simulink model "task5_simulink"  (R2026a)
settings: Solver=VariableStepAuto  StopTime=2
values from neighbouring files (symbols this model uses):
  k = transition_idx(j)    [task4.m]    (also in task5.m = k_values(i); task5_original.m = k_values(i))
  K = place(A, B, desired_poles)    [task3.m]    (also in task4.m; task5.m; task5_original.m)
  x0 = initial_conditions(i,:)'    [task4.m]    (also in task5.m = [0; task5_original.m = [0)
settings Model: Creator=DELL  LastModifiedBy=DELL

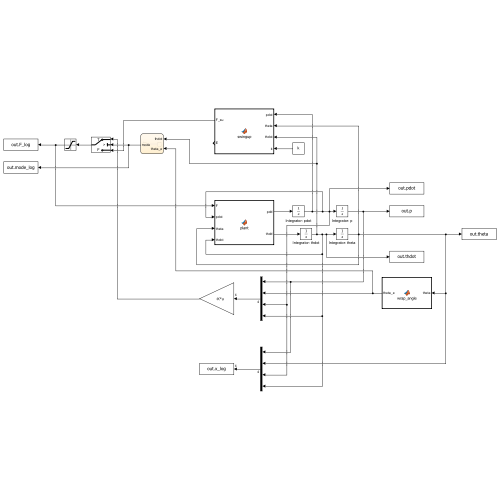
[thumbnail: Simulink's stored preview of the top-level diagram]
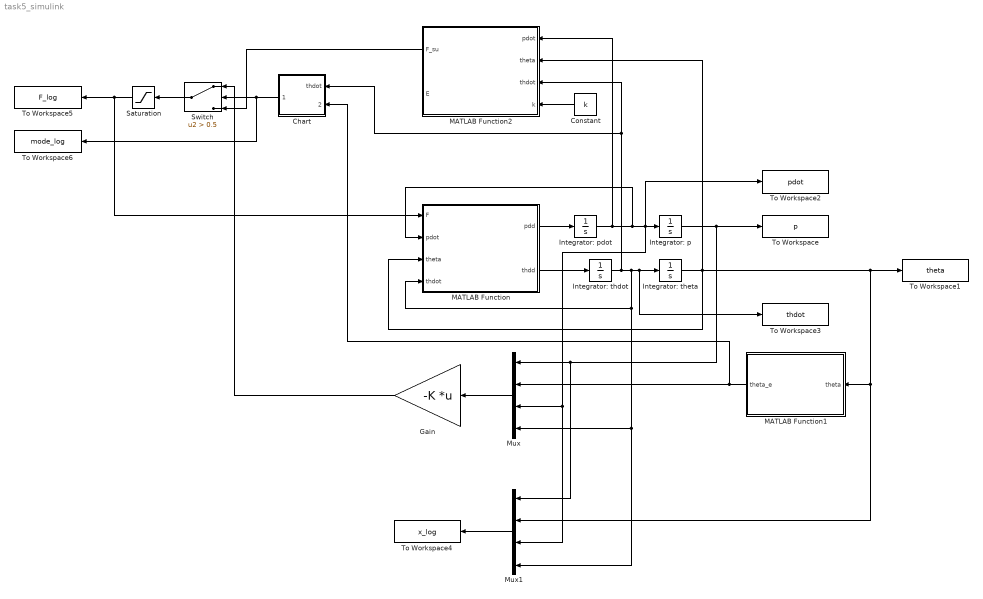
== system task5_simulink ==
  Chart : Stateflow chart  TreatAsAtomicUnit=on
  Constant : Constant  Value=k
  Gain : Gain  Gain=-K  Multiplication=Matrix(K*u)
  Integrator: p : Integrator  InitialCondition=x0(1)
  Integrator: pdot : Integrator  InitialCondition=x0(3)
  Integrator: thdot : Integrator  InitialCondition=x0(4)
  Integrator: theta : Integrator  InitialCondition=x0(2)
  MATLAB Function : MATLAB Function  TreatAsAtomicUnit=on
  MATLAB Function1 : MATLAB Function  TreatAsAtomicUnit=on
  MATLAB Function2 : MATLAB Function  TreatAsAtomicUnit=on
  Mux : Mux
  Mux1 : Mux
  Saturation : Saturate  UpperLimit=14  LowerLimit=-14
  Switch : Switch  Criteria=u2 > Threshold  Threshold=0.5  SaturateOnIntegerOverflow=off  InputSameDT=off
  To Workspace : ToWorkspace  VariableName=p  SaveFormat=Timeseries  SampleTime=0.01
  To Workspace1 : ToWorkspace  VariableName=theta  SaveFormat=Timeseries  SampleTime=0.01
  To Workspace2 : ToWorkspace  VariableName=pdot  SaveFormat=Timeseries  SampleTime=-1
  To Workspace3 : ToWorkspace  VariableName=thdot  SaveFormat=Timeseries  SampleTime=-1
  To Workspace4 : ToWorkspace  VariableName=x_log  SaveFormat=Timeseries  SampleTime=0.01
  To Workspace5 : ToWorkspace  VariableName=F_log  SaveFormat=Timeseries  SampleTime=-1
  To Workspace6 : ToWorkspace  VariableName=mode_log  SaveFormat=Timeseries  SampleTime=-1
  wires:
  MATLAB Function/1(pdd) -> Integrator: pdot/1
  MATLAB Function/2(thdd) -> Integrator: thdot/1
  Integrator: pdot/1 -> MATLAB Function2/1(pdot), MATLAB Function/2(pdot), To Workspace2/1, Integrator: p/1, Mux1/3, Mux/3
  Integrator: thdot/1 -> Chart/1(thdot), MATLAB Function2/3(thdot), Mux1/4, Mux/4, MATLAB Function/4(thdot), To Workspace3/1, Integrator: theta/1
  Integrator: theta/1 -> MATLAB Function2/2(theta), MATLAB Function/3(theta), Mux1/2, MATLAB Function1/1(theta), To Workspace1/1
  Integrator: p/1 -> Mux1/1, Mux/1, To Workspace/1
  Mux/1 -> Gain/1
  Gain/1 -> Switch/1
  MATLAB Function1/1(theta_e) -> Chart/2(theta_e), Mux/2
  Constant/1 -> MATLAB Function2/4(k)
  Chart/1(mode) -> To Workspace6/1, Switch/2
  MATLAB Function2/1(F_su) -> Switch/3
  Switch/1 -> Saturation/1
  Mux1/1 -> To Workspace4/1
  Saturation/1 -> MATLAB Function/1(F), To Workspace5/1

== matlab function task5_simulink/MATLAB Function1 ==
  data: theta input; theta_e output
function theta_e = wrap_angle(theta)

theta_e = atan2(sin(theta), cos(theta));

end

== matlab function task5_simulink/MATLAB Function ==
  data: F input; pdd output; pdot input; theta input; thdot input; thdd output
function [pdd, thdd] = plant(F, pdot, theta, thdot)

M = 5;
m = 1;
l = 0.5;
c = 0.2;
g = 9.8;

pdd = ( ...
    F ...
    - c*pdot ...
    + m*g*sin(theta)*cos(theta) ...
    - m*l*sin(theta)*thdot^2 ...
    ) / (M+m-m*cos(theta)^2);

thdd = ( ...
    cos(theta)*pdd ...
    + g*sin(theta) ...
    ) / l;

end

== matlab function task5_simulink/MATLAB Function2 ==
  data: pdot input; F_su output; theta input; thdot input; k input; E output
function [F_su, E] = swingup(pdot, theta, thdot, k)

M = 5;
m = 1;
l = 0.5;
c = 0.2;
g = 9.8;

E = 0.5*m*l^2*thdot^2 + m*g*l*(cos(theta)-1);
Ed = 0;
beta = 4;

pdd_des = -k*tanh(beta*(E-Ed)*thdot*cos(theta));

D = M + m - m*cos(theta)^2;

F_su = D*pdd_des + c*pdot - m*g*sin(theta)*cos(theta) + m*l*sin(theta)*thdot^2;

end

== stateflow chart task5_simulink/Chart ==
  state SWING_UP
    entry:
    mode = 0;
    during:
    mode = 0;
  state BALANCE
    entry:
    mode = 1;
    during:
    mode = 1;
  (default) -> SWING_UP
  SWING_UP -> BALANCE : [abs(theta_e) < 0.0873 && abs(thdot) < 0.5]
  BALANCE -> SWING_UP : [abs(theta_e) > 0.2618 || abs(thdot) > 1.5]
  data: thdot input; theta_e input; mode output
